simulink model "chapsim"  (R2021b)
settings: Solver=ode45  StartTime=0.0  StopTime=10  RelTol=1e-3  EnableMultiTasking=on
undefined symbols (not defined in the file or in its folder): kd, ki, kp
libraries: simulink_need_slupdate x1
settings Model: Creator=yiyon  LastModifiedBy=yiyon
settings SolverCC: AlgebraicLoopSolver=TrustRegion
settings DataIOCC: SaveFormat=Array  SignalLoggingSaveFormat=ModelDataLogs  ReturnWorkspaceOutputs=off  SignalLoggingName=sigsOut
settings OptimizationCC: BooleanDataType=off  InitFltsAndDblsToZero=on  LifeSpan=inf
settings DebuggingCC: SaveWithParameterizedLinksMsg=none  UnderspecifiedInitializationDetection=Classic  MergeDetectMultiDrivingBlocksExec=none  SignalResolutionControl=TryResolveAllWithWarning  MultiTaskDSMMsg=warning  MultiTaskCondExecSysMsg=none  FcnCallInpInsideContextMsg=warning  SFUnexpectedBacktrackingDiag=warning  SFNoUnconditionalDefaultTransitionDiag=warning  SFExecutionAtInitializationDiag=none  SFMachineParentedDataDiag=warning  ArithmeticOperatorsInVariantConditions=warning
settings HardwareCC: ProdBitPerPointer=32  ProdBitPerSizeT=32  ProdBitPerPtrDiffT=32  ProdLargestAtomicFloat=None  ProdIntDivRoundTo=Undefined  ProdEndianess=Unspecified  ProdWordSize=32  ProdHWDeviceType=32-bit Generic  TargetUnknown=on
settings ModelReferenceCC: PropagateSignalLabelsOutOfModel=off
settings CodeAppCC: StateflowObjectComments=on
settings GRTTargetCC: TargetFcnLib=ansi_tfl_tmw.mat  TargetLangStandard=C89/C90 (ANSI)  CombineOutputUpdateFcns=off  GRTInterface=on
settings ConfigComp: CovMetricSettings=dw  CovSaveCumulativeToWorkspaceVar=on  CovSaveSingleToWorkspaceVar=on

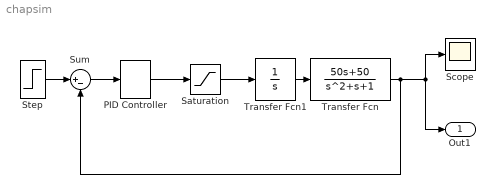
== system chapsim ==
  PID Controller : simulink_need_slupdate/PID Controller  P=kp  I=ki  D=kd
  Saturation : Saturate  UpperLimit=5  LowerLimit=-5
  Scope : Scope
  Step : Step  Time=0  SampleTime=0
  Sum : Sum  Inputs=|+-  InputSameDT=on  SaturateOnIntegerOverflow=on  OutDataTypeStr=Inherit: Same as first input
  Transfer Fcn : TransferFcn  Numerator=[50 50]  Denominator=[1 1 1]
  Transfer Fcn1 : TransferFcn  Denominator=[1 0]
  Out1 : Outport
  wires:
  Sum/1 -> PID Controller/1
  Step/1 -> Sum/1
  Transfer Fcn/1 -> Sum/2, Scope/1, Out1/1
  PID Controller/1 -> Saturation/1
  Transfer Fcn1/1 -> Transfer Fcn/1
  Saturation/1 -> Transfer Fcn1/1
